simulink model "microduck_nonlinear_state_feedback"  (R2026b)
settings: Solver=ode15s  StopTime=r.test.duration  MaxStep=r.p.cfg.sim.maxStep  RelTol=r.p.cfg.sim.relTol  AbsTol=r.p.cfg.sim.absTol
PreLoadFcn:
  | root=fileparts(get_param(bdroot,'FileName')); addpath(root,fullfile(root,'helpers')); md_expanded_cache;
PostLoadFcn:
  | md_sf_apply(bdroot);
InitFcn:
  | md_sf_apply(bdroot);
model workspace (MAT data in the model file):
  G11 = [-0.6  0; 0  -0.6]
  G12 = -12
  G13 = -4000
  G14 = [-0.6  0; 0  -0.6]
  G15 = -12
  G16 = -4000
  G17 = [-0.6  0; 0  -0.6]
  G18 = -12
  G19 = -4000
  G20 = [-0.6  0; 0  -0.6]
  G21 = -12
  G22 = -4000
  G23 = [-0.6  0; 0  -0.6]
  G24 = -12
  G25 = -4000
  G26 = [-0.6  0; 0  -0.6]
  G27 = -12
  G28 = -4000
  G29 = [-0.6  0; 0  -0.6]
  G30 = -12
  G31 = -4000
  G32 = [-0.6  0; 0  -0.6]
  G33 = -12
  G34 = -4000
  G35 = [0 0 0 0 0 0 1 0 0 0 0 0 ... (112 elements, 14x8)]
  G36 = [0 0 0 0 0 0 0.053 0 0 0 0 0 ... (112 elements, 14x8)]
  G39 = [33.3333333333 0 0 0 0 0 0 0 0 33.3333333333 0 0 ... (64 elements, 8x8)]
  G40 = [0 0 0 0 0 0 0 0 0 0 0 0 ... (112 elements, 8x14)]
  G41 = [0 0 0 0 0 0 0 0 0 0 0 0 ... (112 elements, 8x14)]
  Kd_servo = [0 0 0 0 0 0 0 0 0 0 0 0 ... (64 elements, 8x8)]
  Kp_servo = [0.55 0 0 0 0 0 0 0 0 0.55 0 0 ... (64 elements, 8x8)]
  c10 = 0
  c11 = 0
  c13 = 0
  c14 = 0
  c16 = 0
  c17 = 0
  c19 = 0
  c20 = 0
  c22 = 0
  c23 = 0
  c25 = 0
  c26 = 0
  c4 = 0
  c5 = 0
  c7 = 0
  c8 = 0
  g_world = [0; 0; -9.81]
  push_wrench = [1; 0; 0; 0; 0; 0]
  r : object (value not decoded)
  v_s2 = 2.5e-05
symbols that are objects in the model workspace (value not decoded): r
(part 4 of 5)

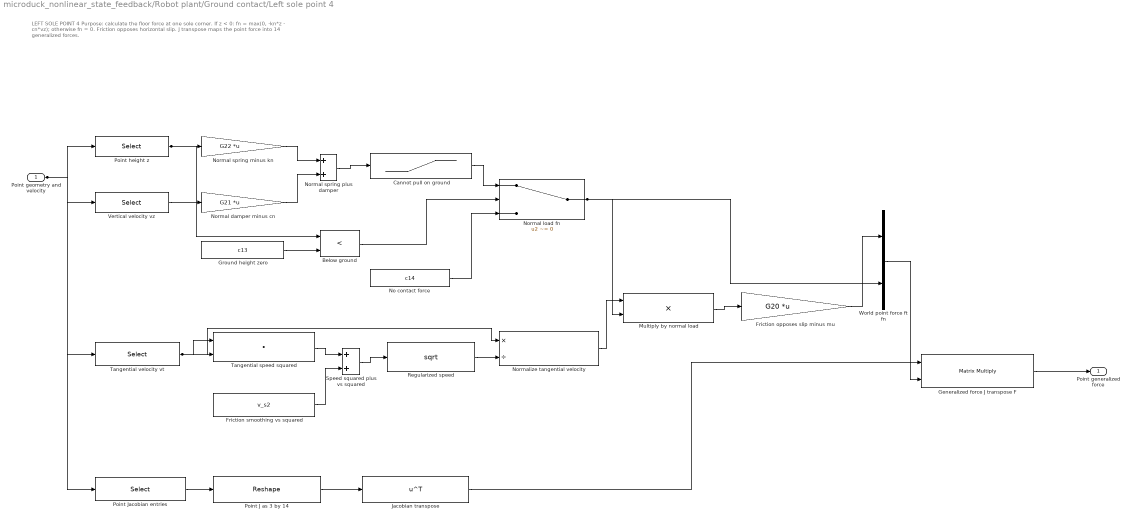
== system microduck_nonlinear_state_feedback/Robot plant/Ground contact/Left sole point 4 ==
  note: LEFT SOLE POINT 4
      |
      | Purpose: calculate the floor force at one sole corner.
      | If z < 0: fn = max(0, -kn*z - cn*vz); otherwise fn = 0.
      | Friction opposes horizontal slip. J transpose maps the point force into 14 generalized forces.
  Point geometry and velocity : Inport  Description=|
      | Point geometry and velocity
      | 
      | WHAT THIS BLOCK DOES
      | Receives this named signal from the parent folder. Check the name for its meaning and units.
      | 
      | FOLDER CONTEXT
      | LEFT SOLE POINT 4
      | 
      | Purpose: calculate the floor force at one sole corner.
      | If z < 0: fn = max(0, -kn*z - cn*vz); otherwise fn = 0.
      | Friction opposes horizontal slip. J transpose maps the point force into 14 generalized forces.
  Below ground : RelationalOperator  Description=|  Operator=<  OutDataTypeStr=boolean  RndMeth=Simplest  InputSameDT=off
      | Below ground
      | 
      | WHAT THIS BLOCK DOES
      | Compares the two inputs. The contact test checks whether the sole point is below the ground plane; true enables normal force.
      | 
      | FOLDER CONTEXT
      | LEFT SOLE POINT 4
      | 
      | Purpose: calculate the floor force at one sole corner.
      | If z < 0: fn = max(0, -kn*z - cn*vz); otherwise fn = 0.
      | Friction opposes horizontal slip. J transpose maps the point force into 14 generalized forces.
  Cannot pull on ground : Saturate  Description=|  UpperLimit=inf  LowerLimit=0
      | Cannot pull on ground
      | 
      | WHAT THIS BLOCK DOES
      | Clips each input element to the permitted interval. Lower bound: 0. Upper bound: inf.
      | 
      | FOLDER CONTEXT
      | LEFT SOLE POINT 4
      | 
      | Purpose: calculate the floor force at one sole corner.
      | If z < 0: fn = max(0, -kn*z - cn*vz); otherwise fn = 0.
      | Friction opposes horizontal slip. J transpose maps the point force into 14 generalized forces.
  Friction opposes slip minus mu : Gain  Description=|  Gain=G20  Multiplication=Matrix(K*u)
      | SHARED PARAMETER: G20 = -r.p.mu*eye(2)
      | Edit sf_parameters.m; per-model edits are refreshed on Run.
      | 
      | WHAT THIS BLOCK DOES
      | Friction opposes slip minus mu
      | 
      | PARAMETER
      | G20 = -r.p.mu*eye(2)
      | 
      | The short symbol is stored in this model workspace. Its numeric value is unchanged from the validated model.
  Friction smoothing vs squared : Constant  Description=|  Value=v_s2
      | SHARED PARAMETER: v_s2 = r.p.vs^2
      | Edit sf_parameters.m; per-model edits are refreshed on Run.
      | 
      | WHAT THIS BLOCK DOES
      | Friction smoothing vs squared
      | 
      | PARAMETER
      | v_s2 = r.p.vs^2
      | 
      | The short symbol is stored in this model workspace. Its numeric value is unchanged from the validated model.
  Generalized force J transpose F : Product  Description=|  Inputs=**  Multiplication=Matrix(*)
      | Generalized force J transpose F
      | 
      | WHAT THIS BLOCK DOES
      | Multiplies/divides the inputs according to the block settings. Input operations: **. The matrix/vector dimensions must agree.
      | 
      | FOLDER CONTEXT
      | LEFT SOLE POINT 4
      | 
      | Purpose: calculate the floor force at one sole corner.
      | If z < 0: fn = max(0, -kn*z - cn*vz); otherwise fn = 0.
      | Friction opposes horizontal slip. J transpose maps the point force into 14 generalized forces.
  Ground height zero : Constant  Description=|  Value=c13
      | SHARED PARAMETER: c13 = 0
      | Edit sf_parameters.m; per-model edits are refreshed on Run.
      | 
      | WHAT THIS BLOCK DOES
      | Ground height zero
      | 
      | PARAMETER
      | c13 = 0
      | 
      | The short symbol is stored in this model workspace. Its numeric value is unchanged from the validated model.
  Jacobian transpose : Math  Description=|  Operator=transpose
      | Jacobian transpose
      | 
      | WHAT THIS BLOCK DOES
      | Performs the mathematical operation named on this block. Open its parameter dialog to inspect the operator and dimensions.
      | 
      | FOLDER CONTEXT
      | LEFT SOLE POINT 4
      | 
      | Purpose: calculate the floor force at one sole corner.
      | If z < 0: fn = max(0, -kn*z - cn*vz); otherwise fn = 0.
      | Friction opposes horizontal slip. J transpose maps the point force into 14 generalized forces.
  Multiply by normal load : Product  Description=|  Inputs=**
      | Multiply by normal load
      | 
      | WHAT THIS BLOCK DOES
      | Multiplies/divides the inputs according to the block settings. Input operations: **. The matrix/vector dimensions must agree.
      | 
      | FOLDER CONTEXT
      | LEFT SOLE POINT 4
      | 
      | Purpose: calculate the floor force at one sole corner.
      | If z < 0: fn = max(0, -kn*z - cn*vz); otherwise fn = 0.
      | Friction opposes horizontal slip. J transpose maps the point force into 14 generalized forces.
  No contact force : Constant  Description=|  Value=c14
      | SHARED PARAMETER: c14 = 0
      | Edit sf_parameters.m; per-model edits are refreshed on Run.
      | 
      | WHAT THIS BLOCK DOES
      | No contact force
      | 
      | PARAMETER
      | c14 = 0
      | 
      | The short symbol is stored in this model workspace. Its numeric value is unchanged from the validated model.
  Normal damper minus cn : Gain  Description=|  Gain=G21  Multiplication=Matrix(K*u)
      | SHARED PARAMETER: G21 = -r.p.cn
      | Edit sf_parameters.m; per-model edits are refreshed on Run.
      | 
      | WHAT THIS BLOCK DOES
      | Normal damper minus cn
      | 
      | PARAMETER
      | G21 = -r.p.cn
      | 
      | The short symbol is stored in this model workspace. Its numeric value is unchanged from the validated model.
  Normal load fn : Switch  Description=|  Criteria=u2 ~= 0  SaturateOnIntegerOverflow=off  InputSameDT=off
      | Normal load fn
      | 
      | WHAT THIS BLOCK DOES
      | Selects the first or third input using the condition on the middle input. For contact, use calculated normal load below ground and zero above ground.
      | 
      | FOLDER CONTEXT
      | LEFT SOLE POINT 4
      | 
      | Purpose: calculate the floor force at one sole corner.
      | If z < 0: fn = max(0, -kn*z - cn*vz); otherwise fn = 0.
      | Friction opposes horizontal slip. J transpose maps the point force into 14 generalized forces.
  Normal spring minus kn : Gain  Description=|  Gain=G22  Multiplication=Matrix(K*u)
      | SHARED PARAMETER: G22 = -r.p.kn
      | Edit sf_parameters.m; per-model edits are refreshed on Run.
      | 
      | WHAT THIS BLOCK DOES
      | Normal spring minus kn
      | 
      | PARAMETER
      | G22 = -r.p.kn
      | 
      | The short symbol is stored in this model workspace. Its numeric value is unchanged from the validated model.
  Normal spring plus damper : Sum  Description=|
      | Normal spring plus damper
      | 
      | WHAT THIS BLOCK DOES
      | Combines its inputs using the plus/minus signs shown on the icon. Signs: ++.
      | 
      | FOLDER CONTEXT
      | LEFT SOLE POINT 4
      | 
      | Purpose: calculate the floor force at one sole corner.
      | If z < 0: fn = max(0, -kn*z - cn*vz); otherwise fn = 0.
      | Friction opposes horizontal slip. J transpose maps the point force into 14 generalized forces.
  Normalize tangential velocity : Product  Description=|  Inputs=*/
      | Normalize tangential velocity
      | 
      | WHAT THIS BLOCK DOES
      | Multiplies/divides the inputs according to the block settings. Input operations: */. The matrix/vector dimensions must agree.
      | 
      | FOLDER CONTEXT
      | LEFT SOLE POINT 4
      | 
      | Purpose: calculate the floor force at one sole corner.
      | If z < 0: fn = max(0, -kn*z - cn*vz); otherwise fn = 0.
      | Friction opposes horizontal slip. J transpose maps the point force into 14 generalized forces.
  Point J as 3 by 14 : Reshape  Description=|  OutputDimensionality=Customize  OutputDimensions=[3 14]
      | Point J as 3 by 14
      | 
      | WHAT THIS BLOCK DOES
      | Changes the arrangement of the entries into the labelled matrix shape. Entries retain MATLAB column-major order and their values do not change.
      | 
      | FOLDER CONTEXT
      | LEFT SOLE POINT 4
      | 
      | Purpose: calculate the floor force at one sole corner.
      | If z < 0: fn = max(0, -kn*z - cn*vz); otherwise fn = 0.
      | Friction opposes horizontal slip. J transpose maps the point force into 14 generalized forces.
  Point Jacobian entries : Selector  Description=|  InputPortWidth=48  IndexOptions=Index vector (dialog)  Indices=[7 8 9 10 11 12 13 14 15 16 17 18 19 20 21 22 23 24 25 26 27 28 29 30 31 32 33 34 35 36 37 38 39 40 41 42 43 44 45 46 47 48]  OutputSizes=1
      | Point Jacobian entries
      | 
      | WHAT THIS BLOCK DOES
      | Selects the labelled coordinates from an input vector without changing their physical values. Open the block to see the one-based index list.
      | 
      | FOLDER CONTEXT
      | LEFT SOLE POINT 4
      | 
      | Purpose: calculate the floor force at one sole corner.
      | If z < 0: fn = max(0, -kn*z - cn*vz); otherwise fn = 0.
      | Friction opposes horizontal slip. J transpose maps the point force into 14 generalized forces.
  Point height z : Selector  Description=|  InputPortWidth=48  IndexOptions=Index vector (dialog)  Indices=3  OutputSizes=1
      | Point height z
      | 
      | WHAT THIS BLOCK DOES
      | Selects the labelled coordinates from an input vector without changing their physical values. Open the block to see the one-based index list.
      | 
      | FOLDER CONTEXT
      | LEFT SOLE POINT 4
      | 
      | Purpose: calculate the floor force at one sole corner.
      | If z < 0: fn = max(0, -kn*z - cn*vz); otherwise fn = 0.
      | Friction opposes horizontal slip. J transpose maps the point force into 14 generalized forces.
  Regularized speed : Math  Description=|  Operator=sqrt
      | Regularized speed
      | 
      | WHAT THIS BLOCK DOES
      | Performs the mathematical operation named on this block. Open its parameter dialog to inspect the operator and dimensions.
      | 
      | FOLDER CONTEXT
      | LEFT SOLE POINT 4
      | 
      | Purpose: calculate the floor force at one sole corner.
      | If z < 0: fn = max(0, -kn*z - cn*vz); otherwise fn = 0.
      | Friction opposes horizontal slip. J transpose maps the point force into 14 generalized forces.
  Speed squared plus vs squared : Sum  Description=|
      | Speed squared plus vs squared
      | 
      | WHAT THIS BLOCK DOES
      | Combines its inputs using the plus/minus signs shown on the icon. Signs: ++.
      | 
      | FOLDER CONTEXT
      | LEFT SOLE POINT 4
      | 
      | Purpose: calculate the floor force at one sole corner.
      | If z < 0: fn = max(0, -kn*z - cn*vz); otherwise fn = 0.
      | Friction opposes horizontal slip. J transpose maps the point force into 14 generalized forces.
  Tangential speed squared : DotProduct  Description=|  OutDataTypeStr=Inherit: Inherit via internal rule
      | Tangential speed squared
      | 
      | WHAT THIS BLOCK DOES
      | Performs the mathematical operation named on this block. Open its parameter dialog to inspect the operator and dimensions.
      | 
      | FOLDER CONTEXT
      | LEFT SOLE POINT 4
      | 
      | Purpose: calculate the floor force at one sole corner.
      | If z < 0: fn = max(0, -kn*z - cn*vz); otherwise fn = 0.
      | Friction opposes horizontal slip. J transpose maps the point force into 14 generalized forces.
  Tangential velocity vt : Selector  Description=|  InputPortWidth=48  IndexOptions=Index vector (dialog)  Indices=[4 5]  OutputSizes=1
      | Tangential velocity vt
      | 
      | WHAT THIS BLOCK DOES
      | Selects the labelled coordinates from an input vector without changing their physical values. Open the block to see the one-based index list.
      | 
      | FOLDER CONTEXT
      | LEFT SOLE POINT 4
      | 
      | Purpose: calculate the floor force at one sole corner.
      | If z < 0: fn = max(0, -kn*z - cn*vz); otherwise fn = 0.
      | Friction opposes horizontal slip. J transpose maps the point force into 14 generalized forces.
  Vertical velocity vz : Selector  Description=|  InputPortWidth=48  IndexOptions=Index vector (dialog)  Indices=6  OutputSizes=1
      | Vertical velocity vz
      | 
      | WHAT THIS BLOCK DOES
      | Selects the labelled coordinates from an input vector without changing their physical values. Open the block to see the one-based index list.
      | 
      | FOLDER CONTEXT
      | LEFT SOLE POINT 4
      | 
      | Purpose: calculate the floor force at one sole corner.
      | If z < 0: fn = max(0, -kn*z - cn*vz); otherwise fn = 0.
      | Friction opposes horizontal slip. J transpose maps the point force into 14 generalized forces.
  World point force ft fn : Mux  Description=|  Inputs=2
      | World point force ft fn
      | 
      | WHAT THIS BLOCK DOES
      | Joins the input vectors in port order, top to bottom. This packages signals; it does not add forces or mix units.
      | 
      | FOLDER CONTEXT
      | LEFT SOLE POINT 4
      | 
      | Purpose: calculate the floor force at one sole corner.
      | If z < 0: fn = max(0, -kn*z - cn*vz); otherwise fn = 0.
      | Friction opposes horizontal slip. J transpose maps the point force into 14 generalized forces.
  Point generalized force : Outport  Description=|
      | Point generalized force
      | 
      | WHAT THIS BLOCK DOES
      | Carries this named result out of the folder. The port number defines the interface order.
      | 
      | FOLDER CONTEXT
      | LEFT SOLE POINT 4
      | 
      | Purpose: calculate the floor force at one sole corner.
      | If z < 0: fn = max(0, -kn*z - cn*vz); otherwise fn = 0.
      | Friction opposes horizontal slip. J transpose maps the point force into 14 generalized forces.
  wires:
  Point height z/1 -> Below ground/1, Normal spring minus kn/1
  Ground height zero/1 -> Below ground/2
  Normal spring plus damper/1 -> Cannot pull on ground/1
  Multiply by normal load/1 -> Friction opposes slip minus mu/1
  Jacobian transpose/1 -> Generalized force J transpose F/1
  World point force ft fn/1 -> Generalized force J transpose F/2
  Point J as 3 by 14/1 -> Jacobian transpose/1
  Normalize tangential velocity/1 -> Multiply by normal load/1
  Normal load fn/1 -> Multiply by normal load/2, World point force ft fn/2
  Vertical velocity vz/1 -> Normal damper minus cn/1
  Cannot pull on ground/1 -> Normal load fn/1
  Below ground/1 -> Normal load fn/2
  No contact force/1 -> Normal load fn/3
  Normal spring minus kn/1 -> Normal spring plus damper/1
  Normal damper minus cn/1 -> Normal spring plus damper/2
  Tangential velocity vt/1 -> Normalize tangential velocity/1, Tangential speed squared/1, Tangential speed squared/2
  Regularized speed/1 -> Normalize tangential velocity/2
  Point Jacobian entries/1 -> Point J as 3 by 14/1
  Point geometry and velocity/1 -> Point Jacobian entries/1, Point height z/1, Tangential velocity vt/1, Vertical velocity vz/1
  Speed squared plus vs squared/1 -> Regularized speed/1
  Tangential speed squared/1 -> Speed squared plus vs squared/1
  Friction smoothing vs squared/1 -> Speed squared plus vs squared/2
  Friction opposes slip minus mu/1 -> World point force ft fn/1
  Generalized force J transpose F/1 -> Point generalized force/1

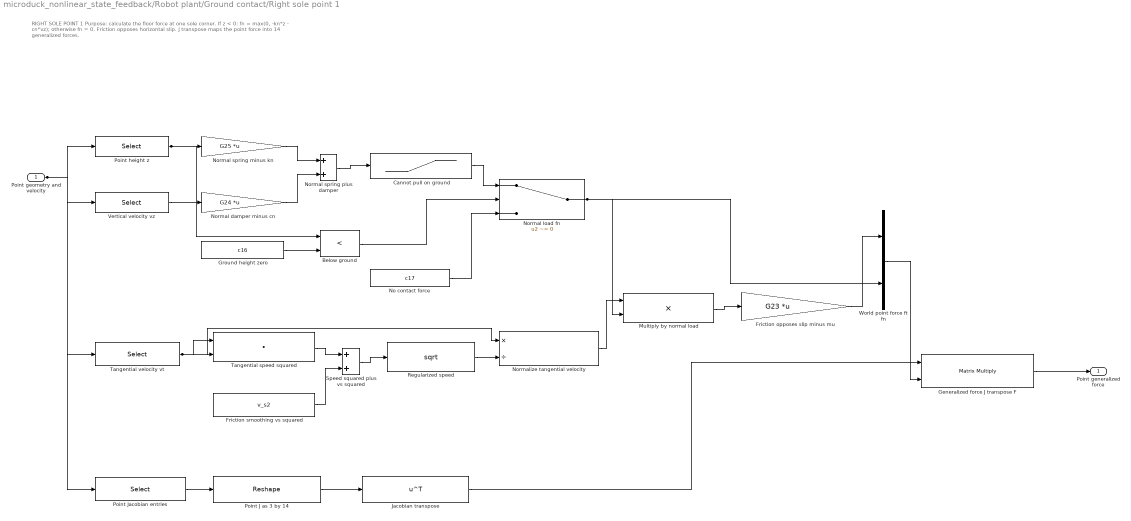
== system microduck_nonlinear_state_feedback/Robot plant/Ground contact/Right sole point 1 ==
  note: RIGHT SOLE POINT 1
      |
      | Purpose: calculate the floor force at one sole corner.
      | If z < 0: fn = max(0, -kn*z - cn*vz); otherwise fn = 0.
      | Friction opposes horizontal slip. J transpose maps the point force into 14 generalized forces.
  Point geometry and velocity : Inport  Description=|
      | Point geometry and velocity
      | 
      | WHAT THIS BLOCK DOES
      | Receives this named signal from the parent folder. Check the name for its meaning and units.
      | 
      | FOLDER CONTEXT
      | RIGHT SOLE POINT 1
      | 
      | Purpose: calculate the floor force at one sole corner.
      | If z < 0: fn = max(0, -kn*z - cn*vz); otherwise fn = 0.
      | Friction opposes horizontal slip. J transpose maps the point force into 14 generalized forces.
  Below ground : RelationalOperator  Description=|  Operator=<  OutDataTypeStr=boolean  RndMeth=Simplest  InputSameDT=off
      | Below ground
      | 
      | WHAT THIS BLOCK DOES
      | Compares the two inputs. The contact test checks whether the sole point is below the ground plane; true enables normal force.
      | 
      | FOLDER CONTEXT
      | RIGHT SOLE POINT 1
      | 
      | Purpose: calculate the floor force at one sole corner.
      | If z < 0: fn = max(0, -kn*z - cn*vz); otherwise fn = 0.
      | Friction opposes horizontal slip. J transpose maps the point force into 14 generalized forces.
  Cannot pull on ground : Saturate  Description=|  UpperLimit=inf  LowerLimit=0
      | Cannot pull on ground
      | 
      | WHAT THIS BLOCK DOES
      | Clips each input element to the permitted interval. Lower bound: 0. Upper bound: inf.
      | 
      | FOLDER CONTEXT
      | RIGHT SOLE POINT 1
      | 
      | Purpose: calculate the floor force at one sole corner.
      | If z < 0: fn = max(0, -kn*z - cn*vz); otherwise fn = 0.
      | Friction opposes horizontal slip. J transpose maps the point force into 14 generalized forces.
  Friction opposes slip minus mu : Gain  Description=|  Gain=G23  Multiplication=Matrix(K*u)
      | SHARED PARAMETER: G23 = -r.p.mu*eye(2)
      | Edit sf_parameters.m; per-model edits are refreshed on Run.
      | 
      | WHAT THIS BLOCK DOES
      | Friction opposes slip minus mu
      | 
      | PARAMETER
      | G23 = -r.p.mu*eye(2)
      | 
      | The short symbol is stored in this model workspace. Its numeric value is unchanged from the validated model.
  Friction smoothing vs squared : Constant  Description=|  Value=v_s2
      | SHARED PARAMETER: v_s2 = r.p.vs^2
      | Edit sf_parameters.m; per-model edits are refreshed on Run.
      | 
      | WHAT THIS BLOCK DOES
      | Friction smoothing vs squared
      | 
      | PARAMETER
      | v_s2 = r.p.vs^2
      | 
      | The short symbol is stored in this model workspace. Its numeric value is unchanged from the validated model.
  Generalized force J transpose F : Product  Description=|  Inputs=**  Multiplication=Matrix(*)
      | Generalized force J transpose F
      | 
      | WHAT THIS BLOCK DOES
      | Multiplies/divides the inputs according to the block settings. Input operations: **. The matrix/vector dimensions must agree.
      | 
      | FOLDER CONTEXT
      | RIGHT SOLE POINT 1
      | 
      | Purpose: calculate the floor force at one sole corner.
      | If z < 0: fn = max(0, -kn*z - cn*vz); otherwise fn = 0.
      | Friction opposes horizontal slip. J transpose maps the point force into 14 generalized forces.
  Ground height zero : Constant  Description=|  Value=c16
      | SHARED PARAMETER: c16 = 0
      | Edit sf_parameters.m; per-model edits are refreshed on Run.
      | 
      | WHAT THIS BLOCK DOES
      | Ground height zero
      | 
      | PARAMETER
      | c16 = 0
      | 
      | The short symbol is stored in this model workspace. Its numeric value is unchanged from the validated model.
  Jacobian transpose : Math  Description=|  Operator=transpose
      | Jacobian transpose
      | 
      | WHAT THIS BLOCK DOES
      | Performs the mathematical operation named on this block. Open its parameter dialog to inspect the operator and dimensions.
      | 
      | FOLDER CONTEXT
      | RIGHT SOLE POINT 1
      | 
      | Purpose: calculate the floor force at one sole corner.
      | If z < 0: fn = max(0, -kn*z - cn*vz); otherwise fn = 0.
      | Friction opposes horizontal slip. J transpose maps the point force into 14 generalized forces.
  Multiply by normal load : Product  Description=|  Inputs=**
      | Multiply by normal load
      | 
      | WHAT THIS BLOCK DOES
      | Multiplies/divides the inputs according to the block settings. Input operations: **. The matrix/vector dimensions must agree.
      | 
      | FOLDER CONTEXT
      | RIGHT SOLE POINT 1
      | 
      | Purpose: calculate the floor force at one sole corner.
      | If z < 0: fn = max(0, -kn*z - cn*vz); otherwise fn = 0.
      | Friction opposes horizontal slip. J transpose maps the point force into 14 generalized forces.
  No contact force : Constant  Description=|  Value=c17
      | SHARED PARAMETER: c17 = 0
      | Edit sf_parameters.m; per-model edits are refreshed on Run.
      | 
      | WHAT THIS BLOCK DOES
      | No contact force
      | 
      | PARAMETER
      | c17 = 0
      | 
      | The short symbol is stored in this model workspace. Its numeric value is unchanged from the validated model.
  Normal damper minus cn : Gain  Description=|  Gain=G24  Multiplication=Matrix(K*u)
      | SHARED PARAMETER: G24 = -r.p.cn
      | Edit sf_parameters.m; per-model edits are refreshed on Run.
      | 
      | WHAT THIS BLOCK DOES
      | Normal damper minus cn
      | 
      | PARAMETER
      | G24 = -r.p.cn
      | 
      | The short symbol is stored in this model workspace. Its numeric value is unchanged from the validated model.
  Normal load fn : Switch  Description=|  Criteria=u2 ~= 0  SaturateOnIntegerOverflow=off  InputSameDT=off
      | Normal load fn
      | 
      | WHAT THIS BLOCK DOES
      | Selects the first or third input using the condition on the middle input. For contact, use calculated normal load below ground and zero above ground.
      | 
      | FOLDER CONTEXT
      | RIGHT SOLE POINT 1
      | 
      | Purpose: calculate the floor force at one sole corner.
      | If z < 0: fn = max(0, -kn*z - cn*vz); otherwise fn = 0.
      | Friction opposes horizontal slip. J transpose maps the point force into 14 generalized forces.
  Normal spring minus kn : Gain  Description=|  Gain=G25  Multiplication=Matrix(K*u)
      | SHARED PARAMETER: G25 = -r.p.kn
      | Edit sf_parameters.m; per-model edits are refreshed on Run.
      | 
      | WHAT THIS BLOCK DOES
      | Normal spring minus kn
      | 
      | PARAMETER
      | G25 = -r.p.kn
      | 
      | The short symbol is stored in this model workspace. Its numeric value is unchanged from the validated model.
  Normal spring plus damper : Sum  Description=|
      | Normal spring plus damper
      | 
      | WHAT THIS BLOCK DOES
      | Combines its inputs using the plus/minus signs shown on the icon. Signs: ++.
      | 
      | FOLDER CONTEXT
      | RIGHT SOLE POINT 1
      | 
      | Purpose: calculate the floor force at one sole corner.
      | If z < 0: fn = max(0, -kn*z - cn*vz); otherwise fn = 0.
      | Friction opposes horizontal slip. J transpose maps the point force into 14 generalized forces.
  Normalize tangential velocity : Product  Description=|  Inputs=*/
      | Normalize tangential velocity
      | 
      | WHAT THIS BLOCK DOES
      | Multiplies/divides the inputs according to the block settings. Input operations: */. The matrix/vector dimensions must agree.
      | 
      | FOLDER CONTEXT
      | RIGHT SOLE POINT 1
      | 
      | Purpose: calculate the floor force at one sole corner.
      | If z < 0: fn = max(0, -kn*z - cn*vz); otherwise fn = 0.
      | Friction opposes horizontal slip. J transpose maps the point force into 14 generalized forces.
  Point J as 3 by 14 : Reshape  Description=|  OutputDimensionality=Customize  OutputDimensions=[3 14]
      | Point J as 3 by 14
      | 
      | WHAT THIS BLOCK DOES
      | Changes the arrangement of the entries into the labelled matrix shape. Entries retain MATLAB column-major order and their values do not change.
      | 
      | FOLDER CONTEXT
      | RIGHT SOLE POINT 1
      | 
      | Purpose: calculate the floor force at one sole corner.
      | If z < 0: fn = max(0, -kn*z - cn*vz); otherwise fn = 0.
      | Friction opposes horizontal slip. J transpose maps the point force into 14 generalized forces.
  Point Jacobian entries : Selector  Description=|  InputPortWidth=48  IndexOptions=Index vector (dialog)  Indices=[7 8 9 10 11 12 13 14 15 16 17 18 19 20 21 22 23 24 25 26 27 28 29 30 31 32 33 34 35 36 37 38 39 40 41 42 43 44 45 46 47 48]  OutputSizes=1
      | Point Jacobian entries
      | 
      | WHAT THIS BLOCK DOES
      | Selects the labelled coordinates from an input vector without changing their physical values. Open the block to see the one-based index list.
      | 
      | FOLDER CONTEXT
      | RIGHT SOLE POINT 1
      | 
      | Purpose: calculate the floor force at one sole corner.
      | If z < 0: fn = max(0, -kn*z - cn*vz); otherwise fn = 0.
      | Friction opposes horizontal slip. J transpose maps the point force into 14 generalized forces.
  Point height z : Selector  Description=|  InputPortWidth=48  IndexOptions=Index vector (dialog)  Indices=3  OutputSizes=1
      | Point height z
      | 
      | WHAT THIS BLOCK DOES
      | Selects the labelled coordinates from an input vector without changing their physical values. Open the block to see the one-based index list.
      | 
      | FOLDER CONTEXT
      | RIGHT SOLE POINT 1
      | 
      | Purpose: calculate the floor force at one sole corner.
      | If z < 0: fn = max(0, -kn*z - cn*vz); otherwise fn = 0.
      | Friction opposes horizontal slip. J transpose maps the point force into 14 generalized forces.
  Regularized speed : Math  Description=|  Operator=sqrt
      | Regularized speed
      | 
      | WHAT THIS BLOCK DOES
      | Performs the mathematical operation named on this block. Open its parameter dialog to inspect the operator and dimensions.
      | 
      | FOLDER CONTEXT
      | RIGHT SOLE POINT 1
      | 
      | Purpose: calculate the floor force at one sole corner.
      | If z < 0: fn = max(0, -kn*z - cn*vz); otherwise fn = 0.
      | Friction opposes horizontal slip. J transpose maps the point force into 14 generalized forces.
  Speed squared plus vs squared : Sum  Description=|
      | Speed squared plus vs squared
      | 
      | WHAT THIS BLOCK DOES
      | Combines its inputs using the plus/minus signs shown on the icon. Signs: ++.
      | 
      | FOLDER CONTEXT
      | RIGHT SOLE POINT 1
      | 
      | Purpose: calculate the floor force at one sole corner.
      | If z < 0: fn = max(0, -kn*z - cn*vz); otherwise fn = 0.
      | Friction opposes horizontal slip. J transpose maps the point force into 14 generalized forces.
  Tangential speed squared : DotProduct  Description=|  OutDataTypeStr=Inherit: Inherit via internal rule
      | Tangential speed squared
      | 
      | WHAT THIS BLOCK DOES
      | Performs the mathematical operation named on this block. Open its parameter dialog to inspect the operator and dimensions.
      | 
      | FOLDER CONTEXT
      | RIGHT SOLE POINT 1
      | 
      | Purpose: calculate the floor force at one sole corner.
      | If z < 0: fn = max(0, -kn*z - cn*vz); otherwise fn = 0.
      | Friction opposes horizontal slip. J transpose maps the point force into 14 generalized forces.
  Tangential velocity vt : Selector  Description=|  InputPortWidth=48  IndexOptions=Index vector (dialog)  Indices=[4 5]  OutputSizes=1
      | Tangential velocity vt
      | 
      | WHAT THIS BLOCK DOES
      | Selects the labelled coordinates from an input vector without changing their physical values. Open the block to see the one-based index list.
      | 
      | FOLDER CONTEXT
      | RIGHT SOLE POINT 1
      | 
      | Purpose: calculate the floor force at one sole corner.
      | If z < 0: fn = max(0, -kn*z - cn*vz); otherwise fn = 0.
      | Friction opposes horizontal slip. J transpose maps the point force into 14 generalized forces.
  Vertical velocity vz : Selector  Description=|  InputPortWidth=48  IndexOptions=Index vector (dialog)  Indices=6  OutputSizes=1
      | Vertical velocity vz
      | 
      | WHAT THIS BLOCK DOES
      | Selects the labelled coordinates from an input vector without changing their physical values. Open the block to see the one-based index list.
      | 
      | FOLDER CONTEXT
      | RIGHT SOLE POINT 1
      | 
      | Purpose: calculate the floor force at one sole corner.
      | If z < 0: fn = max(0, -kn*z - cn*vz); otherwise fn = 0.
      | Friction opposes horizontal slip. J transpose maps the point force into 14 generalized forces.
  World point force ft fn : Mux  Description=|  Inputs=2
      | World point force ft fn
      | 
      | WHAT THIS BLOCK DOES
      | Joins the input vectors in port order, top to bottom. This packages signals; it does not add forces or mix units.
      | 
      | FOLDER CONTEXT
      | RIGHT SOLE POINT 1
      | 
      | Purpose: calculate the floor force at one sole corner.
      | If z < 0: fn = max(0, -kn*z - cn*vz); otherwise fn = 0.
      | Friction opposes horizontal slip. J transpose maps the point force into 14 generalized forces.
  Point generalized force : Outport  Description=|
      | Point generalized force
      | 
      | WHAT THIS BLOCK DOES
      | Carries this named result out of the folder. The port number defines the interface order.
      | 
      | FOLDER CONTEXT
      | RIGHT SOLE POINT 1
      | 
      | Purpose: calculate the floor force at one sole corner.
      | If z < 0: fn = max(0, -kn*z - cn*vz); otherwise fn = 0.
      | Friction opposes horizontal slip. J transpose maps the point force into 14 generalized forces.
  wires:
  Point height z/1 -> Below ground/1, Normal spring minus kn/1
  Ground height zero/1 -> Below ground/2
  Normal spring plus damper/1 -> Cannot pull on ground/1
  Multiply by normal load/1 -> Friction opposes slip minus mu/1
  Jacobian transpose/1 -> Generalized force J transpose F/1
  World point force ft fn/1 -> Generalized force J transpose F/2
  Point J as 3 by 14/1 -> Jacobian transpose/1
  Normalize tangential velocity/1 -> Multiply by normal load/1
  Normal load fn/1 -> Multiply by normal load/2, World point force ft fn/2
  Vertical velocity vz/1 -> Normal damper minus cn/1
  Cannot pull on ground/1 -> Normal load fn/1
  Below ground/1 -> Normal load fn/2
  No contact force/1 -> Normal load fn/3
  Normal spring minus kn/1 -> Normal spring plus damper/1
  Normal damper minus cn/1 -> Normal spring plus damper/2
  Tangential velocity vt/1 -> Normalize tangential velocity/1, Tangential speed squared/1, Tangential speed squared/2
  Regularized speed/1 -> Normalize tangential velocity/2
  Point Jacobian entries/1 -> Point J as 3 by 14/1
  Point geometry and velocity/1 -> Point Jacobian entries/1, Point height z/1, Tangential velocity vt/1, Vertical velocity vz/1
  Speed squared plus vs squared/1 -> Regularized speed/1
  Tangential speed squared/1 -> Speed squared plus vs squared/1
  Friction smoothing vs squared/1 -> Speed squared plus vs squared/2
  Friction opposes slip minus mu/1 -> World point force ft fn/1
  Generalized force J transpose F/1 -> Point generalized force/1

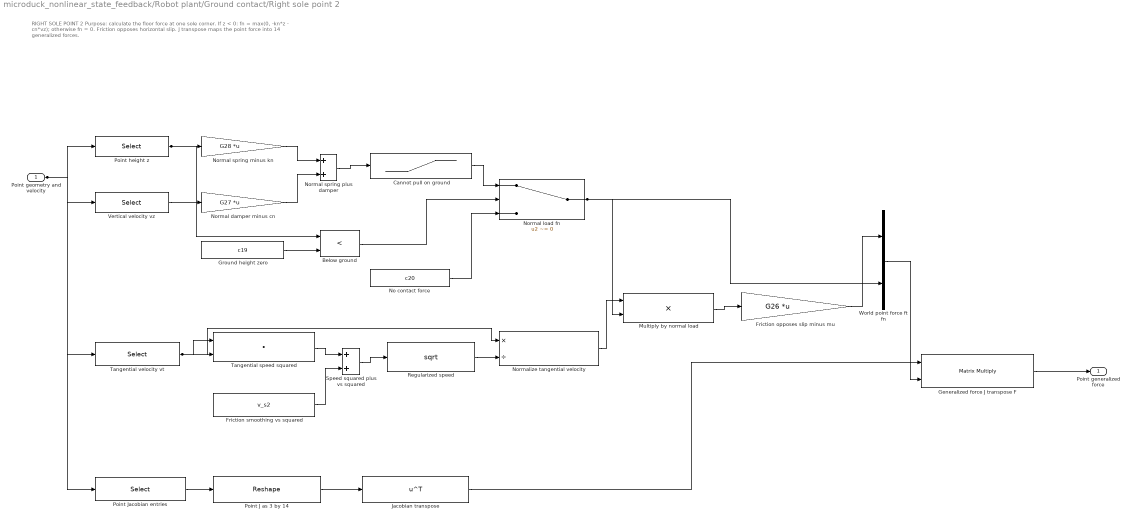
== system microduck_nonlinear_state_feedback/Robot plant/Ground contact/Right sole point 2 ==
  note: RIGHT SOLE POINT 2
      |
      | Purpose: calculate the floor force at one sole corner.
      | If z < 0: fn = max(0, -kn*z - cn*vz); otherwise fn = 0.
      | Friction opposes horizontal slip. J transpose maps the point force into 14 generalized forces.
  Point geometry and velocity : Inport  Description=|
      | Point geometry and velocity
      | 
      | WHAT THIS BLOCK DOES
      | Receives this named signal from the parent folder. Check the name for its meaning and units.
      | 
      | FOLDER CONTEXT
      | RIGHT SOLE POINT 2
      | 
      | Purpose: calculate the floor force at one sole corner.
      | If z < 0: fn = max(0, -kn*z - cn*vz); otherwise fn = 0.
      | Friction opposes horizontal slip. J transpose maps the point force into 14 generalized forces.
  Below ground : RelationalOperator  Description=|  Operator=<  OutDataTypeStr=boolean  RndMeth=Simplest  InputSameDT=off
      | Below ground
      | 
      | WHAT THIS BLOCK DOES
      | Compares the two inputs. The contact test checks whether the sole point is below the ground plane; true enables normal force.
      | 
      | FOLDER CONTEXT
      | RIGHT SOLE POINT 2
      | 
      | Purpose: calculate the floor force at one sole corner.
      | If z < 0: fn = max(0, -kn*z - cn*vz); otherwise fn = 0.
      | Friction opposes horizontal slip. J transpose maps the point force into 14 generalized forces.
  Cannot pull on ground : Saturate  Description=|  UpperLimit=inf  LowerLimit=0
      | Cannot pull on ground
      | 
      | WHAT THIS BLOCK DOES
      | Clips each input element to the permitted interval. Lower bound: 0. Upper bound: inf.
      | 
      | FOLDER CONTEXT
      | RIGHT SOLE POINT 2
      | 
      | Purpose: calculate the floor force at one sole corner.
      | If z < 0: fn = max(0, -kn*z - cn*vz); otherwise fn = 0.
      | Friction opposes horizontal slip. J transpose maps the point force into 14 generalized forces.
  Friction opposes slip minus mu : Gain  Description=|  Gain=G26  Multiplication=Matrix(K*u)
      | SHARED PARAMETER: G26 = -r.p.mu*eye(2)
      | Edit sf_parameters.m; per-model edits are refreshed on Run.
      | 
      | WHAT THIS BLOCK DOES
      | Friction opposes slip minus mu
      | 
      | PARAMETER
      | G26 = -r.p.mu*eye(2)
      | 
      | The short symbol is stored in this model workspace. Its numeric value is unchanged from the validated model.
  Friction smoothing vs squared : Constant  Description=|  Value=v_s2
      | SHARED PARAMETER: v_s2 = r.p.vs^2
      | Edit sf_parameters.m; per-model edits are refreshed on Run.
      | 
      | WHAT THIS BLOCK DOES
      | Friction smoothing vs squared
      | 
      | PARAMETER
      | v_s2 = r.p.vs^2
      | 
      | The short symbol is stored in this model workspace. Its numeric value is unchanged from the validated model.
  Generalized force J transpose F : Product  Description=|  Inputs=**  Multiplication=Matrix(*)
      | Generalized force J transpose F
      | 
      | WHAT THIS BLOCK DOES
      | Multiplies/divides the inputs according to the block settings. Input operations: **. The matrix/vector dimensions must agree.
      | 
      | FOLDER CONTEXT
      | RIGHT SOLE POINT 2
      | 
      | Purpose: calculate the floor force at one sole corner.
      | If z < 0: fn = max(0, -kn*z - cn*vz); otherwise fn = 0.
      | Friction opposes horizontal slip. J transpose maps the point force into 14 generalized forces.
  Ground height zero : Constant  Description=|  Value=c19
      | SHARED PARAMETER: c19 = 0
      | Edit sf_parameters.m; per-model edits are refreshed on Run.
      | 
      | WHAT THIS BLOCK DOES
      | Ground height zero
      | 
      | PARAMETER
      | c19 = 0
      | 
      | The short symbol is stored in this model workspace. Its numeric value is unchanged from the validated model.
  Jacobian transpose : Math  Description=|  Operator=transpose
      | Jacobian transpose
      | 
      | WHAT THIS BLOCK DOES
      | Performs the mathematical operation named on this block. Open its parameter dialog to inspect the operator and dimensions.
      | 
      | FOLDER CONTEXT
      | RIGHT SOLE POINT 2
      | 
      | Purpose: calculate the floor force at one sole corner.
      | If z < 0: fn = max(0, -kn*z - cn*vz); otherwise fn = 0.
      | Friction opposes horizontal slip. J transpose maps the point force into 14 generalized forces.
  Multiply by normal load : Product  Description=|  Inputs=**
      | Multiply by normal load
      | 
      | WHAT THIS BLOCK DOES
      | Multiplies/divides the inputs according to the block settings. Input operations: **. The matrix/vector dimensions must agree.
      | 
      | FOLDER CONTEXT
      | RIGHT SOLE POINT 2
      | 
      | Purpose: calculate the floor force at one sole corner.
      | If z < 0: fn = max(0, -kn*z - cn*vz); otherwise fn = 0.
      | Friction opposes horizontal slip. J transpose maps the point force into 14 generalized forces.
  No contact force : Constant  Description=|  Value=c20
      | SHARED PARAMETER: c20 = 0
      | Edit sf_parameters.m; per-model edits are refreshed on Run.
      | 
      | WHAT THIS BLOCK DOES
      | No contact force
      | 
      | PARAMETER
      | c20 = 0
      | 
      | The short symbol is stored in this model workspace. Its numeric value is unchanged from the validated model.
  Normal damper minus cn : Gain  Description=|  Gain=G27  Multiplication=Matrix(K*u)
      | SHARED PARAMETER: G27 = -r.p.cn
      | Edit sf_parameters.m; per-model edits are refreshed on Run.
      | 
      | WHAT THIS BLOCK DOES
      | Normal damper minus cn
      | 
      | PARAMETER
      | G27 = -r.p.cn
      | 
      | The short symbol is stored in this model workspace. Its numeric value is unchanged from the validated model.
  Normal load fn : Switch  Description=|  Criteria=u2 ~= 0  SaturateOnIntegerOverflow=off  InputSameDT=off
      | Normal load fn
      | 
      | WHAT THIS BLOCK DOES
      | Selects the first or third input using the condition on the middle input. For contact, use calculated normal load below ground and zero above ground.
      | 
      | FOLDER CONTEXT
      | RIGHT SOLE POINT 2
      | 
      | Purpose: calculate the floor force at one sole corner.
      | If z < 0: fn = max(0, -kn*z - cn*vz); otherwise fn = 0.
      | Friction opposes horizontal slip. J transpose maps the point force into 14 generalized forces.
  Normal spring minus kn : Gain  Description=|  Gain=G28  Multiplication=Matrix(K*u)
      | SHARED PARAMETER: G28 = -r.p.kn
      | Edit sf_parameters.m; per-model edits are refreshed on Run.
      | 
      | WHAT THIS BLOCK DOES
      | Normal spring minus kn
      | 
      | PARAMETER
      | G28 = -r.p.kn
      | 
      | The short symbol is stored in this model workspace. Its numeric value is unchanged from the validated model.
  Normal spring plus damper : Sum  Description=|
      | Normal spring plus damper
      | 
      | WHAT THIS BLOCK DOES
      | Combines its inputs using the plus/minus signs shown on the icon. Signs: ++.
      | 
      | FOLDER CONTEXT
      | RIGHT SOLE POINT 2
      | 
      | Purpose: calculate the floor force at one sole corner.
      | If z < 0: fn = max(0, -kn*z - cn*vz); otherwise fn = 0.
      | Friction opposes horizontal slip. J transpose maps the point force into 14 generalized forces.
  Normalize tangential velocity : Product  Description=|  Inputs=*/
      | Normalize tangential velocity
      | 
      | WHAT THIS BLOCK DOES
      | Multiplies/divides the inputs according to the block settings. Input operations: */. The matrix/vector dimensions must agree.
      | 
      | FOLDER CONTEXT
      | RIGHT SOLE POINT 2
      | 
      | Purpose: calculate the floor force at one sole corner.
      | If z < 0: fn = max(0, -kn*z - cn*vz); otherwise fn = 0.
      | Friction opposes horizontal slip. J transpose maps the point force into 14 generalized forces.
  Point J as 3 by 14 : Reshape  Description=|  OutputDimensionality=Customize  OutputDimensions=[3 14]
      | Point J as 3 by 14
      | 
      | WHAT THIS BLOCK DOES
      | Changes the arrangement of the entries into the labelled matrix shape. Entries retain MATLAB column-major order and their values do not change.
      | 
      | FOLDER CONTEXT
      | RIGHT SOLE POINT 2
      | 
      | Purpose: calculate the floor force at one sole corner.
      | If z < 0: fn = max(0, -kn*z - cn*vz); otherwise fn = 0.
      | Friction opposes horizontal slip. J transpose maps the point force into 14 generalized forces.
  Point Jacobian entries : Selector  Description=|  InputPortWidth=48  IndexOptions=Index vector (dialog)  Indices=[7 8 9 10 11 12 13 14 15 16 17 18 19 20 21 22 23 24 25 26 27 28 29 30 31 32 33 34 35 36 37 38 39 40 41 42 43 44 45 46 47 48]  OutputSizes=1
      | Point Jacobian entries
      | 
      | WHAT THIS BLOCK DOES
      | Selects the labelled coordinates from an input vector without changing their physical values. Open the block to see the one-based index list.
      | 
      | FOLDER CONTEXT
      | RIGHT SOLE POINT 2
      | 
      | Purpose: calculate the floor force at one sole corner.
      | If z < 0: fn = max(0, -kn*z - cn*vz); otherwise fn = 0.
      | Friction opposes horizontal slip. J transpose maps the point force into 14 generalized forces.
  Point height z : Selector  Description=|  InputPortWidth=48  IndexOptions=Index vector (dialog)  Indices=3  OutputSizes=1
      | Point height z
      | 
      | WHAT THIS BLOCK DOES
      | Selects the labelled coordinates from an input vector without changing their physical values. Open the block to see the one-based index list.
      | 
      | FOLDER CONTEXT
      | RIGHT SOLE POINT 2
      | 
      | Purpose: calculate the floor force at one sole corner.
      | If z < 0: fn = max(0, -kn*z - cn*vz); otherwise fn = 0.
      | Friction opposes horizontal slip. J transpose maps the point force into 14 generalized forces.
  Regularized speed : Math  Description=|  Operator=sqrt
      | Regularized speed
      | 
      | WHAT THIS BLOCK DOES
      | Performs the mathematical operation named on this block. Open its parameter dialog to inspect the operator and dimensions.
      | 
      | FOLDER CONTEXT
      | RIGHT SOLE POINT 2
      | 
      | Purpose: calculate the floor force at one sole corner.
      | If z < 0: fn = max(0, -kn*z - cn*vz); otherwise fn = 0.
      | Friction opposes horizontal slip. J transpose maps the point force into 14 generalized forces.
  Speed squared plus vs squared : Sum  Description=|
      | Speed squared plus vs squared
      | 
      | WHAT THIS BLOCK DOES
      | Combines its inputs using the plus/minus signs shown on the icon. Signs: ++.
      | 
      | FOLDER CONTEXT
      | RIGHT SOLE POINT 2
      | 
      | Purpose: calculate the floor force at one sole corner.
      | If z < 0: fn = max(0, -kn*z - cn*vz); otherwise fn = 0.
      | Friction opposes horizontal slip. J transpose maps the point force into 14 generalized forces.
  Tangential speed squared : DotProduct  Description=|  OutDataTypeStr=Inherit: Inherit via internal rule
      | Tangential speed squared
      | 
      | WHAT THIS BLOCK DOES
      | Performs the mathematical operation named on this block. Open its parameter dialog to inspect the operator and dimensions.
      | 
      | FOLDER CONTEXT
      | RIGHT SOLE POINT 2
      | 
      | Purpose: calculate the floor force at one sole corner.
      | If z < 0: fn = max(0, -kn*z - cn*vz); otherwise fn = 0.
      | Friction opposes horizontal slip. J transpose maps the point force into 14 generalized forces.
  Tangential velocity vt : Selector  Description=|  InputPortWidth=48  IndexOptions=Index vector (dialog)  Indices=[4 5]  OutputSizes=1
      | Tangential velocity vt
      | 
      | WHAT THIS BLOCK DOES
      | Selects the labelled coordinates from an input vector without changing their physical values. Open the block to see the one-based index list.
      | 
      | FOLDER CONTEXT
      | RIGHT SOLE POINT 2
      | 
      | Purpose: calculate the floor force at one sole corner.
      | If z < 0: fn = max(0, -kn*z - cn*vz); otherwise fn = 0.
      | Friction opposes horizontal slip. J transpose maps the point force into 14 generalized forces.
  Vertical velocity vz : Selector  Description=|  InputPortWidth=48  IndexOptions=Index vector (dialog)  Indices=6  OutputSizes=1
      | Vertical velocity vz
      | 
      | WHAT THIS BLOCK DOES
      | Selects the labelled coordinates from an input vector without changing their physical values. Open the block to see the one-based index list.
      | 
      | FOLDER CONTEXT
      | RIGHT SOLE POINT 2
      | 
      | Purpose: calculate the floor force at one sole corner.
      | If z < 0: fn = max(0, -kn*z - cn*vz); otherwise fn = 0.
      | Friction opposes horizontal slip. J transpose maps the point force into 14 generalized forces.
  World point force ft fn : Mux  Description=|  Inputs=2
      | World point force ft fn
      | 
      | WHAT THIS BLOCK DOES
      | Joins the input vectors in port order, top to bottom. This packages signals; it does not add forces or mix units.
      | 
      | FOLDER CONTEXT
      | RIGHT SOLE POINT 2
      | 
      | Purpose: calculate the floor force at one sole corner.
      | If z < 0: fn = max(0, -kn*z - cn*vz); otherwise fn = 0.
      | Friction opposes horizontal slip. J transpose maps the point force into 14 generalized forces.
  Point generalized force : Outport  Description=|
      | Point generalized force
      | 
      | WHAT THIS BLOCK DOES
      | Carries this named result out of the folder. The port number defines the interface order.
      | 
      | FOLDER CONTEXT
      | RIGHT SOLE POINT 2
      | 
      | Purpose: calculate the floor force at one sole corner.
      | If z < 0: fn = max(0, -kn*z - cn*vz); otherwise fn = 0.
      | Friction opposes horizontal slip. J transpose maps the point force into 14 generalized forces.
  wires:
  Point height z/1 -> Below ground/1, Normal spring minus kn/1
  Ground height zero/1 -> Below ground/2
  Normal spring plus damper/1 -> Cannot pull on ground/1
  Multiply by normal load/1 -> Friction opposes slip minus mu/1
  Jacobian transpose/1 -> Generalized force J transpose F/1
  World point force ft fn/1 -> Generalized force J transpose F/2
  Point J as 3 by 14/1 -> Jacobian transpose/1
  Normalize tangential velocity/1 -> Multiply by normal load/1
  Normal load fn/1 -> Multiply by normal load/2, World point force ft fn/2
  Vertical velocity vz/1 -> Normal damper minus cn/1
  Cannot pull on ground/1 -> Normal load fn/1
  Below ground/1 -> Normal load fn/2
  No contact force/1 -> Normal load fn/3
  Normal spring minus kn/1 -> Normal spring plus damper/1
  Normal damper minus cn/1 -> Normal spring plus damper/2
  Tangential velocity vt/1 -> Normalize tangential velocity/1, Tangential speed squared/1, Tangential speed squared/2
  Regularized speed/1 -> Normalize tangential velocity/2
  Point Jacobian entries/1 -> Point J as 3 by 14/1
  Point geometry and velocity/1 -> Point Jacobian entries/1, Point height z/1, Tangential velocity vt/1, Vertical velocity vz/1
  Speed squared plus vs squared/1 -> Regularized speed/1
  Tangential speed squared/1 -> Speed squared plus vs squared/1
  Friction smoothing vs squared/1 -> Speed squared plus vs squared/2
  Friction opposes slip minus mu/1 -> World point force ft fn/1
  Generalized force J transpose F/1 -> Point generalized force/1
